simulink model "SIS4"  (R2023a)
settings: Solver=ode15s  StartTime=0.0  StopTime=10  MaxStep=1E-3  RelTol=1e-3
libraries: fl_lib x14, nesl_utility x6, slpidlib x1
settings Model: Creator=cdhan  LastModifiedBy=MSI
settings DataIOCC: SaveOutput=off  SignalLogging=off  DSMLogging=off  ReturnWorkspaceOutputs=off  TimeSaveName=t
settings DebuggingCC: AlgebraicLoopMsg=none  ArtificialAlgebraicLoopMsg=none  MaxConsecutiveZCsMsg=none  ModelReferenceExtraNoncontSigs=none  OperatingPointInterfaceChecksumMismatchMsg=none

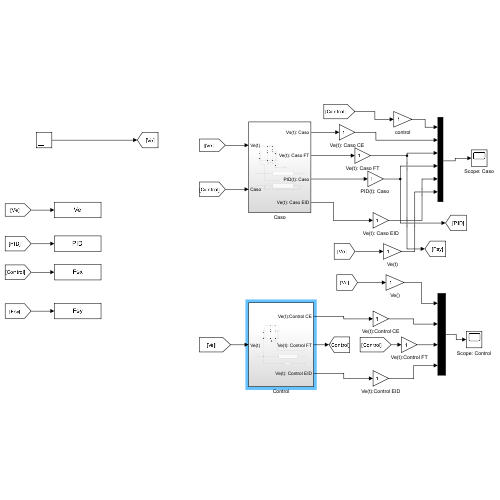
[thumbnail: Simulink's stored preview of the top-level diagram]
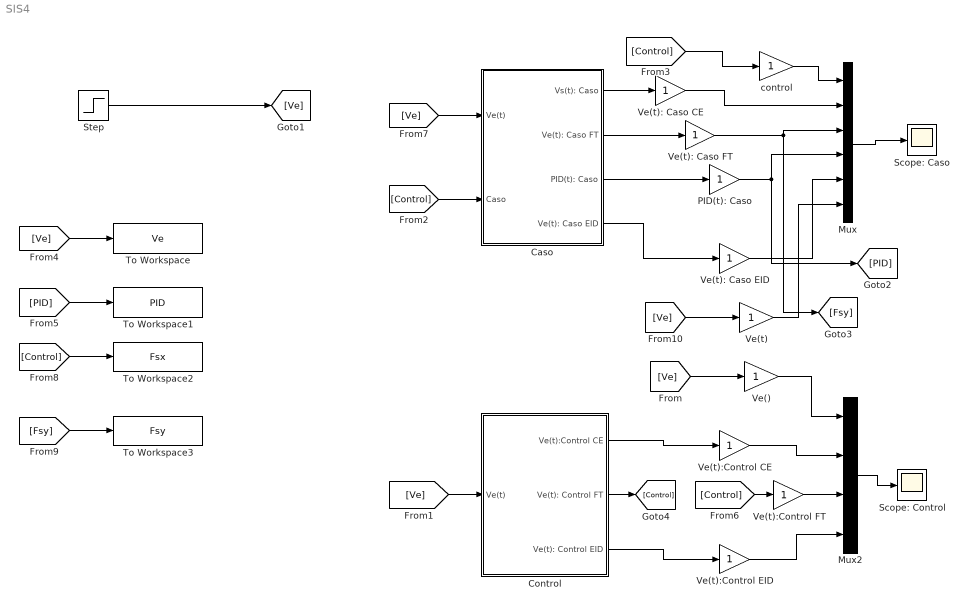
== system SIS4 ==
  Caso : Subsystem
  Control : Subsystem
  Mux : Mux  Inputs=6
  Mux2 : Mux
  "PID(t): Caso " : Gain
  Scope: Caso : Scope
  Scope: Control : Scope
  Step : Step  Time=0  SampleTime=0
  To Workspace : ToWorkspace  VariableName=Ve  SampleTime=-1
  To Workspace1 : ToWorkspace  VariableName=PID  SampleTime=-1
  To Workspace2 : ToWorkspace  VariableName=Fsx  SampleTime=-1
  To Workspace3 : ToWorkspace  VariableName=Fsy  SampleTime=-1
  Ve() : Gain
  Ve(t) : Gain
  Ve(t): Caso CE : Gain
  Ve(t): Caso EID : Gain
  Ve(t): Caso FT : Gain
  Ve(t):Control CE : Gain
  Ve(t):Control EID : Gain
  Ve(t):Control FT : Gain
  control : Gain
  wires:
  "PID(t): Caso "/1 -> [PID], Mux/4
  Ve(t): Caso FT/1 -> [Fsy], Mux/3
  Caso/2(Ve(t): Caso FT) -> Ve(t): Caso FT/1
  [Ve] -> Control/1(Ve(t))
  Mux/1 -> Scope: Caso/1
  [Control] -> Caso/2(Caso)
  Ve(t): Caso CE/1 -> Mux/2
  Caso/1(Vs(t): Caso) -> Ve(t): Caso CE/1
  Control/2(Ve(t): Control FT) -> [Control]
  Mux2/1 -> Scope: Control/1
  [Ve] -> Caso/1(Ve(t))
  [Control] -> Ve(t):Control FT/1
  Control/1(Ve(t):Control CE) -> Ve(t):Control CE/1
  Step/1 -> [Ve]
  Caso/3(PID(t): Caso) -> "PID(t): Caso "/1
  Control/3(Ve(t): Control EID) -> Ve(t):Control EID/1
  Caso/4(Ve(t): Caso EID) -> Ve(t): Caso EID/1
  Ve(t): Caso EID/1 -> Mux/5
  control/1 -> Mux/1
  [Control] -> control/1
  Ve(t):Control EID/1 -> Mux2/4
  Ve(t):Control FT/1 -> Mux2/3
  Ve(t):Control CE/1 -> Mux2/2
  [Ve] -> Ve()/1
  Ve()/1 -> Mux2/1
  [Ve] -> To Workspace/1
  [PID] -> To Workspace1/1
  [Control] -> To Workspace2/1
  [Fsy] -> To Workspace3/1
  [Ve] -> Ve(t)/1
  Ve(t)/1 -> Mux/6

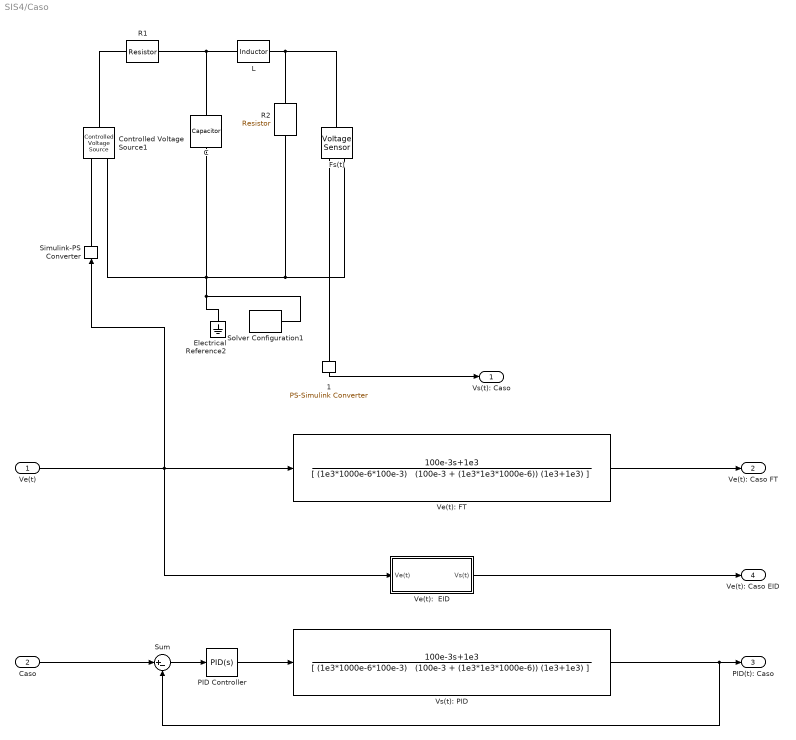
== system SIS4/Caso ==
  Ve(t) : Inport
  Caso : Inport  Port=2
  1 : nesl_utility/PS-Simulink Converter  PhysicalDomain=network_engine_domain  SubClassName=ps_output  LeftPortType=input  RightPortType=output  PseudoPeriodic=off  Frequencies=[]  VectorFormat=1-D array  Unit=inherit  AffineConversion=off
  C : fl_lib/Electrical/Electrical Elements/Capacitor  c=1000 uF  r=1e-6 Ohm  g=0 1/Ohm  i_specify=off  i_priority=None  i=0 A  i_nominal_specify=off  i_nominal_unit=A  i_nominal_value=1  v_specify=off  v_priority=None  v=0 V  v_nominal_specify=off  v_nominal_unit=V  v_nominal_value=1  vc_specify=off  vc_priority=High  vc=0 V  vc_nominal_specify=off  vc_nominal_unit=V  vc_nominal_value=1
  Controlled Voltage Source1 : fl_lib/Electrical/Electrical Sources/Controlled Voltage Source
  Electrical Reference2 : fl_lib/Electrical/Electrical Elements/Electrical Reference
  Fs(t) : fl_lib/Electrical/Electrical Sensors/Voltage Sensor
  L : fl_lib/Electrical/Electrical Elements/Inductor  l=100 mH  r=0 Ohm  g=1e-9 1/Ohm  i_specify=off  i_priority=None  i=0 A  i_nominal_specify=off  i_nominal_unit=A  i_nominal_value=1  v_specify=off  v_priority=None  v=0 V  v_nominal_specify=off  v_nominal_unit=V  v_nominal_value=1  i_L_specify=off  i_L_priority=High  i_L=0 A  i_L_nominal_specify=off  i_L_nominal_unit=A  i_L_nominal_value=1
  PID Controller : slpidlib/PID Controller  Controller=PID  Form=Parallel  TimeDomain=Continuous-time  UseExternalTs=off  SampleTime=-1  IntegratorMethod=Forward Euler  FilterMethod=Forward Euler  ControllerParametersSource=internal  P=529.0879  I=51836.0493  UseKiTs=off  D=0.17756  N=2021.2211  UseFilter=on  TunerSelectOption=Transfer Function Based (PID Tuner App)  InitialConditionSource=internal  InitialConditionForIntegrator=0  InitialConditionForFilter=0  DifferentiatorICPrevScaledInput=0  ExternalReset=none  TrackingMode=off  Kt=1  LimitOutput=off  SatLimitsSource=internal  UpperSaturationLimit=inf  LowerSaturationLimit=-inf  LinearizeAsGain=on  AntiWindupMode=none  Kb=1  LimitIntegrator=off  UpperIntegratorSaturationLimit=inf  LowerIntegratorSaturationLimit=-inf  POutMin=[]  POutMax=[]  IOutMin=[]  IOutMax=[]  DOutMin=[]  DOutMax=[]  NOutMin=[]  NOutMax=[]  SumOutMin=[]  SumOutMax=[]  SaturationOutMin=[]  SaturationOutMax=[]  PParamMin=[]  PParamMax=[]  IParamMin=[]  IParamMax=[]  DParamMin=[]  DParamMax=[]  NParamMin=[]  NParamMax=[]  KbParamMin=[]  KbParamMax=[]  KtParamMin=[]  KtParamMax=[]  KbOutMin=[]  KbOutMax=[]  KtOutMin=[]  KtOutMax=[]  IntegratorOutMin=[]  IntegratorOutMax=[]  FilterOutMin=[]  FilterOutMax=[]  SumI1OutMin=[]  SumI1OutMax=[]  SumI2OutMin=[]  SumI2OutMax=[]  SumI3OutMin=[]  SumI3OutMax=[]  SumI4OutMin=[]  SumI4OutMax=[]  SumDOutMin=[]  SumDOutMax=[]  DifferentiatorOutMin=[]  DifferentiatorOutMax=[]  FilterDiffOutCoefMin=[]  FilterDiffOutCoefMax=[]  ReciprocalOutMin=[]  ReciprocalOutMax=[]  SumDenOutMin=[]  SumDenOutMax=[]  SumNumOutMin=[]  SumNumOutMax=[]  DivideOutMin=[]  DivideOutMax=[]  UdiffTsProdOutMin=[]  UdiffTsProdOutMax=[]  NTsProdOutMin=[]  NTsProdOutMax=[]  UintegralTsProdOutMin=[]  UintegralTsProdOutMax=[]  UngainTsProdOutMin=[]  UngainTsProdOutMax=[]  ClampingZeroOutDataTypeStr=Inherit: Inherit via back propagation  ClampingZeroOutMin=[]  ClampingZeroOutMax=[]  FilterDenConstantOutDataTypeStr=Inherit: Inherit via back propagation  FilterDenConstantOutMin=[]  FilterDenConstantOutMax=[]  PCopyOutDataTypeStr=Inherit: Inherit via back propagation  PCopyOutMin=[]  PCopyOutMax=[]  NCopyOutDataTypeStr=Inherit: Inherit via back propagation  NCopyOutMin=[]  NCopyOutMax=[]  IntegratorContinuousStateAttributes=''  IntegratorStateMustResolveToSignalObject=off  IntegratorRTWStateStorageClass=Auto  FilterContinuousStateAttributes=''  FilterStateMustResolveToSignalObject=off  FilterRTWStateStorageClass=Auto  ParallelPVariant=InternalParameters  IdealPVariant=Disabled  IVariant=InternalParameters  DVariant=InternalParameters  IntegratorVariant=Continuous  SatVariant=Disabled  AWVariant=Passthrough  PCopyVariant=Disabled  TRVariant=Disabled  FdbkBlocksVariant=Forward  IdealPFdbkVariant=Disabled  SatFdbkVariant=Disabled  DerivativeFilterVariant=ContFilter  NVariant=InternalParameters  NCopyVariant=Disabled  FilterICVariant=InternalICsFilter  IntegratorICVariant=InternalICs  ExternalResetVariant=Disabled  TRSumVariant=Passthrough  SumFdbkVariant=Disabled  SumVariant=Sum_PID  TsampFilterVariant=InternalTs  TsampNgainVariant=Passthrough  TsampIntegralVariant=Disabled_SignalSpec  ExternalSaturationOutDataTypeStr=Inherit: Same as second input
  R1 : fl_lib/Electrical/Electrical Elements/Resistor  R=1 kOhm  i_specify=off  i_priority=None  i=0 A  i_nominal_specify=off  i_nominal_unit=A  i_nominal_value=1  v_specify=off  v_priority=None  v=0 V  v_nominal_specify=off  v_nominal_unit=V  v_nominal_value=1
  R2 : fl_lib/Electrical/Electrical Elements/Resistor  R=1 kOhm  i_specify=off  i_priority=None  i=0 A  i_nominal_specify=off  i_nominal_unit=A  i_nominal_value=1  v_specify=off  v_priority=None  v=0 V  v_nominal_specify=off  v_nominal_unit=V  v_nominal_value=1
  Simulink-PS Converter : nesl_utility/Simulink-PS Converter  PhysicalDomain=network_engine_domain  SubClassName=ps_input  LeftPortType=input  RightPortType=output  PseudoPeriodic=off  Frequencies=[]  NoiseDistribution=none  NoiseParameters=[]  Unit=1  AffineConversion=off  FilteringAndDerivatives=provide  SimscapeFilterOrder=1  InputFilterTimeConstant=0.001  UdotUserProvided=0
  Solver Configuration1 : nesl_utility/Solver Configuration  PhysicalDomain=network_engine_domain  SubClassName=solver  LeftPortType=input  RightPortType=generic  Tones=[]  Harmonics=[]  SimulateNoise=off  Profile=off  UseLocalSampling=off  EnableSwitchedLinearOptims=on  FrequencyDomain=off  UseCCode=off  RelTol=0.001  AbsTol=0.001  MinStep=1e-09  ToWorkspace=off  RevertToSquareIcSolve=off  NumHomotopyIterations=100  PhasorMode=off  PhasorModeNumHarmonics=1  ConsistencySolver=NEWTON_XTOL_AFTER_FTOL  IndexReductionMethod=DerivativeReplacement  DoDC=off  ResidualTolerance=1e-09  ConsistencyTolSource=GLOBAL  ConsistencyAbsTol=0.001  ConsistencyRelTol=0.001  ConsistencyTolFactor=0.001  UseLocalSolver=off  LocalSolverChoice=NE_BACKWARD_EULER_ADVANCER  ResolveIndetEquations=on  FunctionEvalNumThread=1  LocalSolverSampleTime=0.001  DoFixedCost=off  MaxNonlinIter=3  MaxModeIter=2  ComputeImpulses=off  ImpulseIterations=2  LinearAlgebra=auto  LinearAlgebraNumThread=0  EquationFormulation=NE_TIME_EF  DelaysMemoryBudget=1024  AutomaticFiltering=on  FilteringTimeConstant=0.001  PartitionStorageMethod=AS_NEEDED  PartitionMemoryBudget=1024  PartitionMethod=ROBUST
  Sum : Sum  Inputs=|+-
  Ve(t):  EID : Subsystem
  Ve(t): FT : TransferFcn  Numerator=[100e-3, 1e3]  Denominator="[ (1e3*1000e-6*100e-3)   (100e-3 + (1e3*1e3*1000e-6)) (1e3+1e3) ]"
  Vs(t): PID : TransferFcn  Numerator=[100e-3, 1e3]  Denominator="[ (1e3*1000e-6*100e-3)   (100e-3 + (1e3*1e3*1000e-6)) (1e3+1e3) ]"
  Vs(t): Caso : Outport
  Ve(t): Caso FT : Outport  Port=2
  PID(t): Caso : Outport  Port=3
  Ve(t): Caso EID : Outport  Port=4
  wires:
  Sum/1 -> PID Controller/1
  PID Controller/1 -> Vs(t): PID/1
  Vs(t): PID/1 -> PID(t): Caso/1, Sum/2
  Ve(t)/1 -> Ve(t):  EID/1(Ve(t)), Simulink-PS Converter/1, Ve(t): FT/1
  Ve(t): FT/1 -> Ve(t): Caso FT/1
  Caso/1 -> Sum/1
  1/1 -> Vs(t): Caso/1
  Ve(t):  EID/1(Vs(t)) -> Ve(t): Caso EID/1
  connections:
  L/LConn1 -- R1/LConn1 -- C/LConn1
  Controlled Voltage Source1/RConn2 -- R2/LConn1 -- Fs(t)/RConn2 -- Electrical Reference2/LConn1 -- Solver Configuration1/RConn1 -- C/RConn1
  Controlled Voltage Source1/LConn1 -- R1/RConn1
  Controlled Voltage Source1/RConn1 -- Simulink-PS Converter/RConn1
  Fs(t)/RConn1 -- 1/LConn1
  L/RConn1 -- Fs(t)/LConn1 -- R2/RConn1

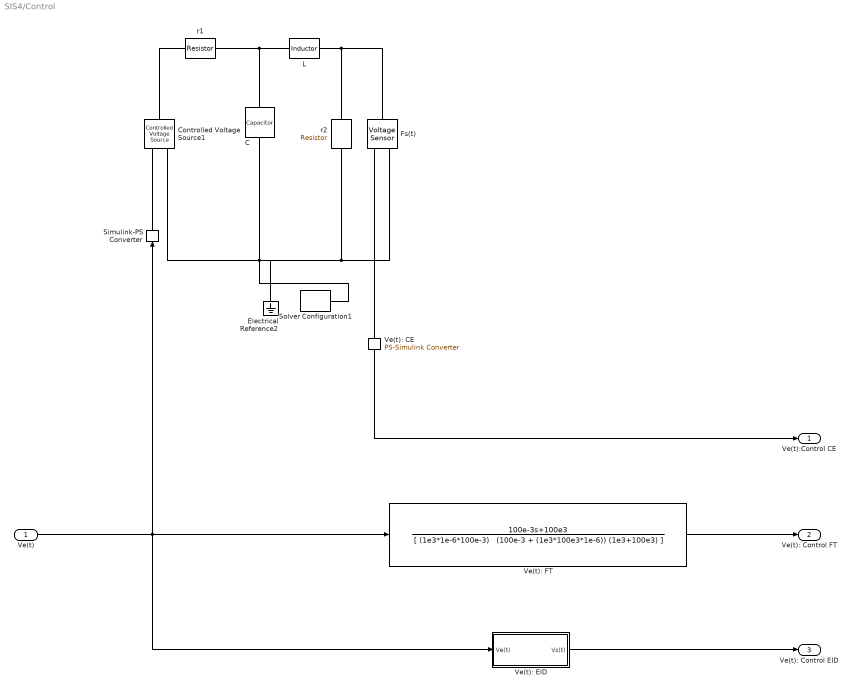
== system SIS4/Control ==
  Ve(t) : Inport
  C : fl_lib/Electrical/Electrical Elements/Capacitor  c=1 uF  r=1e-6 Ohm  g=0 1/Ohm  i_specify=off  i_priority=None  i=0 A  i_nominal_specify=off  i_nominal_unit=A  i_nominal_value=1  v_specify=off  v_priority=None  v=0 V  v_nominal_specify=off  v_nominal_unit=V  v_nominal_value=1  vc_specify=off  vc_priority=High  vc=0 V  vc_nominal_specify=off  vc_nominal_unit=V  vc_nominal_value=1
  Controlled Voltage Source1 : fl_lib/Electrical/Electrical Sources/Controlled Voltage Source
  Electrical Reference2 : fl_lib/Electrical/Electrical Elements/Electrical Reference
  Fs(t) : fl_lib/Electrical/Electrical Sensors/Voltage Sensor
  L : fl_lib/Electrical/Electrical Elements/Inductor  l=100 mH  r=0 Ohm  g=1e-9 1/Ohm  i_specify=off  i_priority=None  i=0 A  i_nominal_specify=off  i_nominal_unit=A  i_nominal_value=1  v_specify=off  v_priority=None  v=0 V  v_nominal_specify=off  v_nominal_unit=V  v_nominal_value=1  i_L_specify=off  i_L_priority=High  i_L=0 A  i_L_nominal_specify=off  i_L_nominal_unit=A  i_L_nominal_value=1
  Simulink-PS Converter : nesl_utility/Simulink-PS Converter  PhysicalDomain=network_engine_domain  SubClassName=ps_input  LeftPortType=input  RightPortType=output  PseudoPeriodic=off  Frequencies=[]  NoiseDistribution=none  NoiseParameters=[]  Unit=1  AffineConversion=off  FilteringAndDerivatives=provide  SimscapeFilterOrder=1  InputFilterTimeConstant=0.001  UdotUserProvided=0
  Solver Configuration1 : nesl_utility/Solver Configuration  PhysicalDomain=network_engine_domain  SubClassName=solver  LeftPortType=input  RightPortType=generic  Tones=[]  Harmonics=[]  SimulateNoise=off  Profile=off  UseLocalSampling=off  EnableSwitchedLinearOptims=on  FrequencyDomain=off  UseCCode=off  RelTol=0.001  AbsTol=0.001  MinStep=1e-09  ToWorkspace=off  RevertToSquareIcSolve=off  NumHomotopyIterations=100  PhasorMode=off  PhasorModeNumHarmonics=1  ConsistencySolver=NEWTON_XTOL_AFTER_FTOL  IndexReductionMethod=DerivativeReplacement  DoDC=off  ResidualTolerance=1e-09  ConsistencyTolSource=GLOBAL  ConsistencyAbsTol=0.001  ConsistencyRelTol=0.001  ConsistencyTolFactor=0.001  UseLocalSolver=off  LocalSolverChoice=NE_BACKWARD_EULER_ADVANCER  ResolveIndetEquations=on  FunctionEvalNumThread=1  LocalSolverSampleTime=0.001  DoFixedCost=off  MaxNonlinIter=3  MaxModeIter=2  ComputeImpulses=off  ImpulseIterations=2  LinearAlgebra=auto  LinearAlgebraNumThread=0  EquationFormulation=NE_TIME_EF  DelaysMemoryBudget=1024  AutomaticFiltering=on  FilteringTimeConstant=0.001  PartitionStorageMethod=AS_NEEDED  PartitionMemoryBudget=1024  PartitionMethod=ROBUST
  Ve(t): CE : nesl_utility/PS-Simulink Converter  PhysicalDomain=network_engine_domain  SubClassName=ps_output  LeftPortType=input  RightPortType=output  PseudoPeriodic=off  Frequencies=[]  VectorFormat=1-D array  Unit=inherit  AffineConversion=off
  Ve(t): EID : Subsystem
  Ve(t): FT : TransferFcn  Numerator=[100e-3, 100e3]  Denominator="[ (1e3*1e-6*100e-3)   (100e-3 + (1e3*100e3*1e-6)) (1e3+100e3) ]"
  r1 : fl_lib/Electrical/Electrical Elements/Resistor  R=1 kOhm  i_specify=off  i_priority=None  i=0 A  i_nominal_specify=off  i_nominal_unit=A  i_nominal_value=1  v_specify=off  v_priority=None  v=0 V  v_nominal_specify=off  v_nominal_unit=V  v_nominal_value=1
  r2 : fl_lib/Electrical/Electrical Elements/Resistor  R=100 kOhm  i_specify=off  i_priority=None  i=0 A  i_nominal_specify=off  i_nominal_unit=A  i_nominal_value=1  v_specify=off  v_priority=None  v=0 V  v_nominal_specify=off  v_nominal_unit=V  v_nominal_value=1
  Ve(t):Control CE : Outport
  Ve(t): Control FT : Outport  Port=2
  Ve(t): Control EID : Outport  Port=3
  wires:
  Ve(t)/1 -> Ve(t): EID/1(Ve(t)), Simulink-PS Converter/1, Ve(t): FT/1
  Ve(t): FT/1 -> Ve(t): Control FT/1
  Ve(t): CE/1 -> Ve(t):Control CE/1
  Ve(t): EID/1(Vs(t)) -> Ve(t): Control EID/1
  connections:
  Controlled Voltage Source1/RConn1 -- Simulink-PS Converter/RConn1
  Fs(t)/RConn1 -- Ve(t): CE/LConn1
  Fs(t)/RConn2 -- Solver Configuration1/RConn1 -- Electrical Reference2/LConn1 -- C/RConn1 -- Controlled Voltage Source1/RConn2 -- r2/LConn1
  Controlled Voltage Source1/LConn1 -- r1/RConn1
  r1/LConn1 -- C/LConn1 -- L/LConn1
  r2/RConn1 -- Fs(t)/LConn1 -- L/RConn1

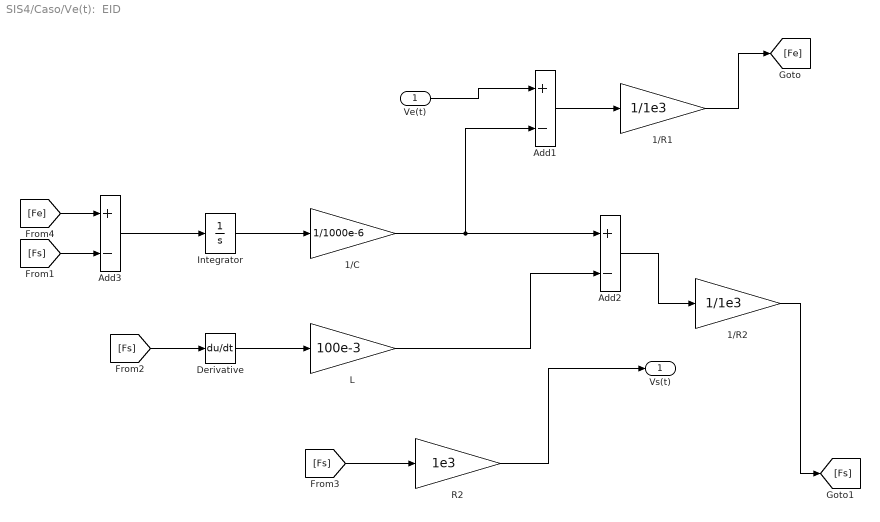
== system SIS4/Caso/Ve(t):  EID ==
  Ve(t) : Inport
  1/C : Gain  Gain=1/1000e-6
  1/R1 : Gain  Gain=1/1e3
  1/R2 : Gain  Gain=1/1e3
  Add1 : Sum  Inputs=+-
  Add2 : Sum  Inputs=+-
  Add3 : Sum  Inputs=+-
  Derivative : Derivative
  Integrator : Integrator
  L : Gain  Gain=100e-3
  R2 : Gain  Gain=1e3
  Vs(t) : Outport
  wires:
  [Fe] -> Add3/1
  [Fs] -> Add3/2
  Ve(t)/1 -> Add1/1
  Add3/1 -> Integrator/1
  Integrator/1 -> 1/C/1
  1/C/1 -> Add1/2, Add2/1
  Derivative/1 -> L/1
  [Fs] -> Derivative/1
  L/1 -> Add2/2
  [Fs] -> R2/1
  Add1/1 -> 1/R1/1
  1/R1/1 -> [Fe]
  Add2/1 -> 1/R2/1
  R2/1 -> Vs(t)/1
  1/R2/1 -> [Fs]

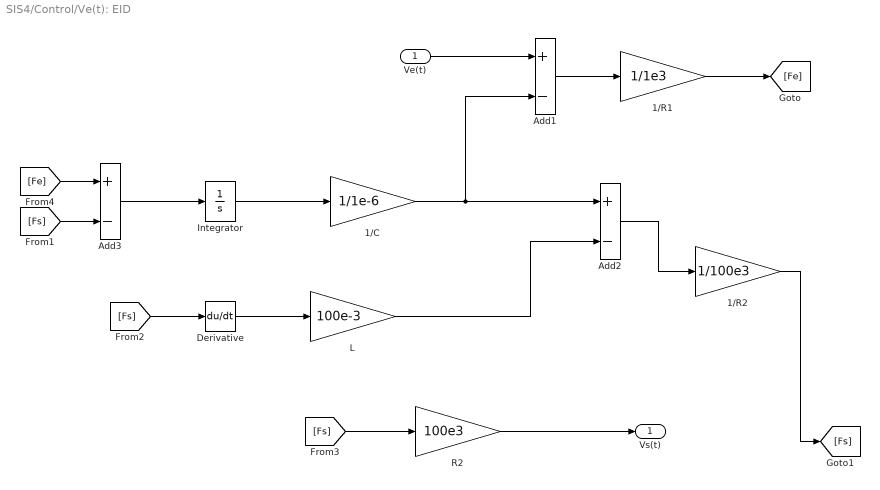
== system SIS4/Control/Ve(t): EID ==
  Ve(t) : Inport
  1/C : Gain  Gain=1/1e-6
  1/R1 : Gain  Gain=1/1e3
  1/R2 : Gain  Gain=1/100e3
  Add1 : Sum  Inputs=+-
  Add2 : Sum  Inputs=+-
  Add3 : Sum  Inputs=+-
  Derivative : Derivative
  Integrator : Integrator
  L : Gain  Gain=100e-3
  R2 : Gain  Gain=100e3
  Vs(t) : Outport
  wires:
  [Fe] -> Add3/1
  [Fs] -> Add3/2
  Ve(t)/1 -> Add1/1
  Add3/1 -> Integrator/1
  Integrator/1 -> 1/C/1
  1/C/1 -> Add1/2, Add2/1
  Derivative/1 -> L/1
  [Fs] -> Derivative/1
  L/1 -> Add2/2
  [Fs] -> R2/1
  Add1/1 -> 1/R1/1
  1/R1/1 -> [Fe]
  Add2/1 -> 1/R2/1
  R2/1 -> Vs(t)/1
  1/R2/1 -> [Fs]
